simulink model "bus_hvac"  (R2025a)
settings: Solver=VariableStepAuto  StartTime=0.0  StopTime=7200  MaxStep=1  RelTol=1e-3
PreLoadFcn:
  | bus_hvac_params
InitFcn:
  | if ~exist('T_set', 'var'), bus_hvac_params; end
values from neighbouring files (symbols this model uses):
  blow_set = [42 38 28 22]    [bus_hvac_params.m]
  blow_T = [-20 0 10 18]    [bus_hvac_params.m]
  C_cab = cab_mass_factor*rho_air*V_cab*cp_air    (= 361800)    [bus_hvac_params.m]
  c_w = 3600    [bus_hvac_params.m]
  cp_air = 1005    [bus_hvac_params.m]
  d_fan1_off = 0.02    [bus_hvac_params.m]
  d_fan1_on = 0.05    [bus_hvac_params.m]
  d_fan2_off = 0.3    [bus_hvac_params.m]
  d_fan2_on = 0.9    [bus_hvac_params.m]
  d_on = 0.02    [bus_hvac_params.m]
  der_f = [1 1 0.6]    [bus_hvac_params.m]
  der_T = [-40 55 90]    [bus_hvac_params.m]
  e_cool_off = -0.3    [bus_hvac_params.m]
  e_cool_on = 0.5    [bus_hvac_params.m]
  e_heat_off = -0.5    [bus_hvac_params.m]
  e_heat_on = 0.3    [bus_hvac_params.m]
  e_heater_off = -8    [bus_hvac_params.m]
  e_heater_on = 2    [bus_hvac_params.m]
  EER = 2.5    [bus_hvac_params.m]
  eps_front = 0.7    [bus_hvac_params.m]
  front_fan = 1    [bus_hvac_params.m]
  front_margin = 15    [bus_hvac_params.m]
  fuel_enable = 0    [bus_hvac_params.m]
  G_byp = 1/sqrt(K_byp)    [bus_hvac_params.m]
  G_grid = linspace(G_byp, Gc_tab(end) + Gf_tab(end) + G_byp, 30)    [bus_hvac_params.m]
  Gc_tab = 1./sqrt(K_conv + K_valve./h_grid.^2)    [bus_hvac_params.m]
  Gf_tab = 1./sqrt(K_front + K_valve./h_grid.^2)    [bus_hvac_params.m]
  h_grid = linspace(valve_min, 1, 20)    [bus_hvac_params.m]
  hp_COP = [1.6 2.0 2.6 3.2 3.6]    [bus_hvac_params.m]
  hp_enable = 1    [bus_hvac_params.m]
  hp_Qheat = [8000 12000 16000 18000 18000]    [bus_hvac_params.m]
  hp_T = [-20 -10 0 10 20]    [bus_hvac_params.m]
  Ki_cab = 0.004    [bus_hvac_params.m]
  Ki_f = 0.002    [bus_hvac_params.m]
  Ki_h = 0.002    [bus_hvac_params.m]
  Ki_v = 0.0015    [bus_hvac_params.m]
  Kp_f = 0.05    [bus_hvac_params.m]
  Kp_h = 0.08    [bus_hvac_params.m]
  Kp_v = 0.08    [bus_hvac_params.m]
  m_air_front = 0.25    [bus_hvac_params.m]
  M_aux = 8    [bus_hvac_params.m]
  M_conv = 20    [bus_hvac_params.m]
  M_fhx = 1.5    [bus_hvac_params.m]
  m_flow_min = 0.05    [bus_hvac_params.m]
  m_fresh = 0.10    (= 0.1)    [bus_hvac_params.m]
  M_fret = 4    [bus_hvac_params.m]
  M_fsup = 4    [bus_hvac_params.m]
  M_heater = 3    [bus_hvac_params.m]
  mar = [15 10 5]    [bus_hvac_params.m]
  mar_T = [-20 0 15]    [bus_hvac_params.m]
  mtot_tab = sqrt(dp0./(b_pump + K_src + 1./G_grid.^2))    [bus_hvac_params.m]
  n_pass = 20    [bus_hvac_params.m]
  P_fuel_max = 30000    [bus_hvac_params.m]
  P_heater_max = 20000    [bus_hvac_params.m]
  P_pump = 150    [bus_hvac_params.m]
  Q_cool_max = 20000    [bus_hvac_params.m]
  q_pass = 75    [bus_hvac_params.m]
  Q_solar = 0    [bus_hvac_params.m]
  T_cab0 = -10    [bus_hvac_params.m]
  T_conv_max = 65    [bus_hvac_params.m]
  T_cool_lock = 12    [bus_hvac_params.m]
  t_dwell = 300    [bus_hvac_params.m]
  T_fan_off = 35    [bus_hvac_params.m]
  T_fan_on = 40    [bus_hvac_params.m]
  T_fuel_cut = 85    [bus_hvac_params.m]
  t_fuel_ignite = 60    [bus_hvac_params.m]
  T_fuel_off = 78    [bus_hvac_params.m]
  T_fuel_on = 65    [bus_hvac_params.m]
  T_fuel_out_max = 5    [bus_hvac_params.m]
  T_heat_lock = 18    [bus_hvac_params.m]
  T_heater_cut = 88    [bus_hvac_params.m]
  T_heater_cut_hyst = 10    [bus_hvac_params.m]
  t_heater_delay = 10    [bus_hvac_params.m]
  T_out_time = [0 7200]    [bus_hvac_params.m]
  T_out_val = [-10 -10]    [bus_hvac_params.m]
  t_pump_run = 60    [bus_hvac_params.m]
  T_set = 22    [bus_hvac_params.m]
  T_sup_max = 85    [bus_hvac_params.m]
  T_w0 = -10    [bus_hvac_params.m]
  tau_fuel = 60    [bus_hvac_params.m]
  Ts_mode = 5    [bus_hvac_params.m]
  UA_cab = U_wall*A_wall + U_glass*A_glass    (= 222.4)    [bus_hvac_params.m]
  UA_conv_stage = [30 130 220]    [bus_hvac_params.m]
  valve_min = 0.05    [bus_hvac_params.m]
undefined symbols (not defined in the file or in its folder): Kp_cab
settings Model: Creator=giray  LastModifiedBy=giray

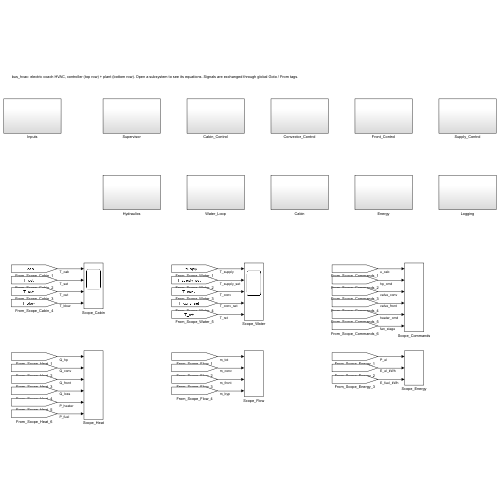
[thumbnail: Simulink's stored preview of the top-level diagram]
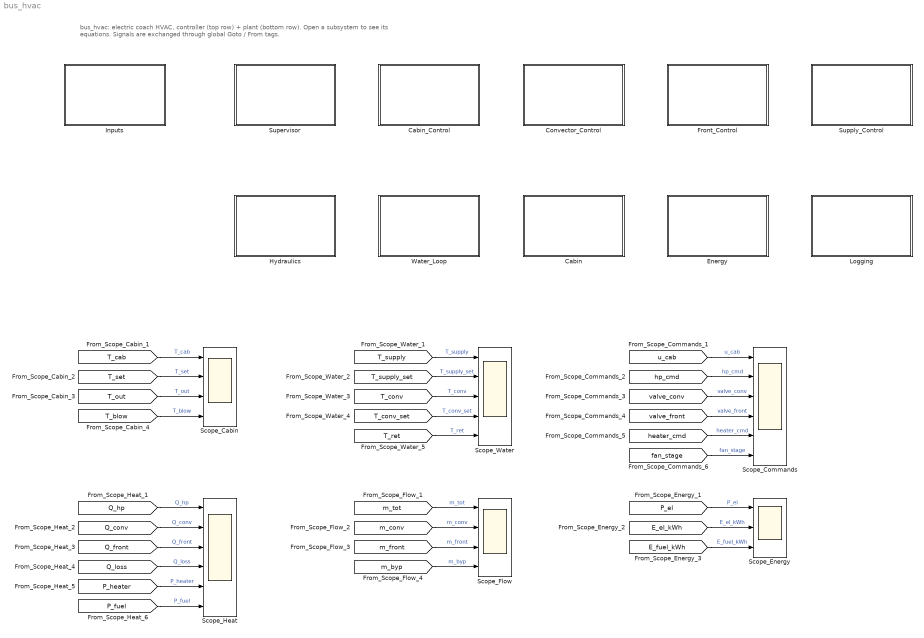
== system bus_hvac ==
  note: bus_hvac: electric coach HVAC, controller (top row) + plant (bottom row). Open a subsystem to see its equations. Signals are exchanged through global Goto / From tags.
  Cabin : Subsystem
  Cabin_Control : Subsystem
  Convector_Control : Subsystem
  Energy : Subsystem
  Front_Control : Subsystem
  Hydraulics : Subsystem
  Inputs : Subsystem
  Logging : Subsystem
  Scope_Cabin : Scope  NumInputPorts=4
  Scope_Commands : Scope  NumInputPorts=6
  Scope_Energy : Scope  NumInputPorts=3
  Scope_Flow : Scope  NumInputPorts=4
  Scope_Heat : Scope  NumInputPorts=6
  Scope_Water : Scope  NumInputPorts=5
  Supervisor : Subsystem
  Supply_Control : Subsystem
  Water_Loop : Subsystem
  wires:
  [T_cab] -> Scope_Cabin/1  "T_cab"
  [T_set] -> Scope_Cabin/2  "T_set"
  [T_out] -> Scope_Cabin/3  "T_out"
  [T_blow] -> Scope_Cabin/4  "T_blow"
  [T_supply] -> Scope_Water/1  "T_supply"
  [T_supply_set] -> Scope_Water/2  "T_supply_set"
  [T_conv] -> Scope_Water/3  "T_conv"
  [T_conv_set] -> Scope_Water/4  "T_conv_set"
  [T_ret] -> Scope_Water/5  "T_ret"
  [u_cab] -> Scope_Commands/1  "u_cab"
  [hp_cmd] -> Scope_Commands/2  "hp_cmd"
  [valve_conv] -> Scope_Commands/3  "valve_conv"
  [valve_front] -> Scope_Commands/4  "valve_front"
  [heater_cmd] -> Scope_Commands/5  "heater_cmd"
  [fan_stage] -> Scope_Commands/6  "fan_stage"
  [Q_hp] -> Scope_Heat/1  "Q_hp"
  [Q_conv] -> Scope_Heat/2  "Q_conv"
  [Q_front] -> Scope_Heat/3  "Q_front"
  [Q_loss] -> Scope_Heat/4  "Q_loss"
  [P_heater] -> Scope_Heat/5  "P_heater"
  [P_fuel] -> Scope_Heat/6  "P_fuel"
  [m_tot] -> Scope_Flow/1  "m_tot"
  [m_conv] -> Scope_Flow/2  "m_conv"
  [m_front] -> Scope_Flow/3  "m_front"
  [m_byp] -> Scope_Flow/4  "m_byp"
  [P_el] -> Scope_Energy/1  "P_el"
  [E_el_kWh] -> Scope_Energy/2  "E_el_kWh"
  [E_fuel_kWh] -> Scope_Energy/3  "E_fuel_kWh"

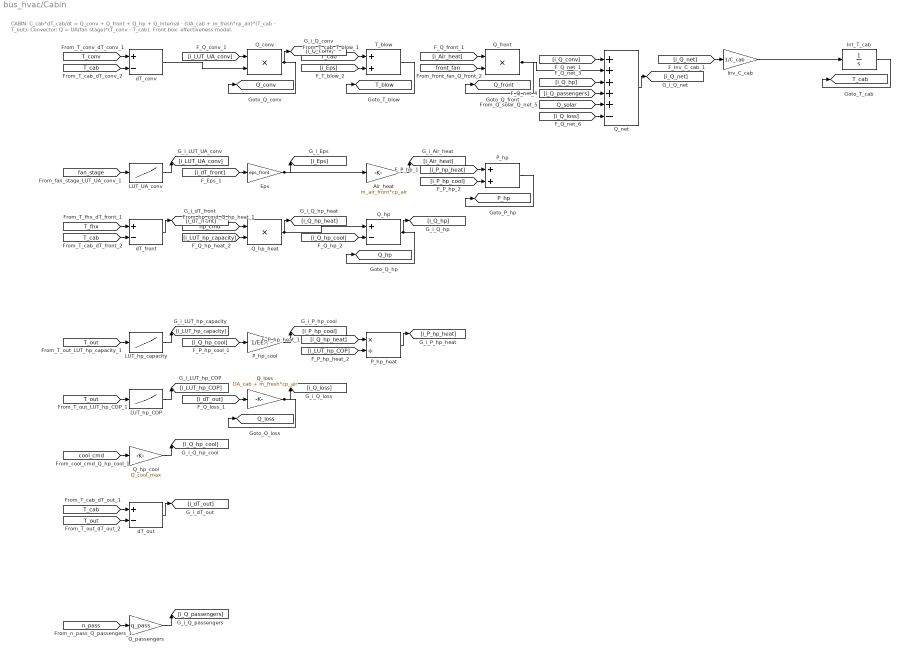
== system bus_hvac/Cabin ==
  note: CABIN: C_cab*dT_cab/dt = Q_conv + Q_front + Q_hp + Q_internal - (UA_cab + m_fresh*cp_air)*(T_cab - T_out). Convector: Q = UA(fan stage)*(T_conv - T_cab). Front box: effectiveness model.
  Air_heat : Gain  Gain=m_air_front*cp_air
  Eps : Gain  Gain=eps_front
  Int_T_cab : Integrator  InitialCondition=T_cab0
  Inv_C_cab : Gain  Gain=1/C_cab
  LUT_UA_conv : Lookup_n-D  NumberOfTableDimensions=1  BreakpointsForDimension1=[0 1 2]  Table=UA_conv_stage  ExtrapMethod=Clip  InternalRulePriority=Speed  RndMeth=Simplest
  LUT_hp_COP : Lookup_n-D  NumberOfTableDimensions=1  BreakpointsForDimension1=hp_T  Table=hp_COP  ExtrapMethod=Clip  InternalRulePriority=Speed  RndMeth=Simplest
  LUT_hp_capacity : Lookup_n-D  NumberOfTableDimensions=1  BreakpointsForDimension1=hp_T  Table=hp_Qheat  ExtrapMethod=Clip  InternalRulePriority=Speed  RndMeth=Simplest
  P_hp : Sum
  P_hp_cool : Gain  Gain=1/EER
  P_hp_heat : Product  Inputs=*/
  Q_conv : Product
  Q_front : Product
  Q_hp : Sum  Inputs=+-
  Q_hp_cool : Gain  Gain=Q_cool_max
  Q_hp_heat : Product
  Q_loss : Gain  Gain=UA_cab + m_fresh*cp_air
  Q_net : Sum  Inputs=+++++-
  Q_passengers : Gain  Gain=q_pass
  T_blow : Sum
  dT_conv : Sum  Inputs=+-
  dT_front : Sum  Inputs=+-
  dT_out : Sum  Inputs=+-
  tag scope: P_hp=global, Q_conv=global, Q_front=global, Q_hp=global, Q_loss=global, T_blow=global, T_cab=global
  wires:
  [T_conv] -> dT_conv/1
  [T_cab] -> dT_conv/2
  [fan_stage] -> LUT_UA_conv/1
  LUT_UA_conv/1 -> [i_LUT_UA_conv]
  [i_LUT_UA_conv] -> Q_conv/1
  dT_conv/1 -> Q_conv/2
  [T_fhx] -> dT_front/1
  [T_cab] -> dT_front/2
  dT_front/1 -> [i_dT_front]
  [i_dT_front] -> Eps/1
  [T_cab] -> T_blow/1
  Eps/1 -> [i_Eps], Air_heat/1
  [i_Eps] -> T_blow/2
  Air_heat/1 -> [i_Air_heat]
  [i_Air_heat] -> Q_front/1
  [front_fan] -> Q_front/2
  [T_out] -> LUT_hp_capacity/1
  [T_out] -> LUT_hp_COP/1
  [hp_cmd] -> Q_hp_heat/1
  LUT_hp_capacity/1 -> [i_LUT_hp_capacity]
  [i_LUT_hp_capacity] -> Q_hp_heat/2
  [cool_cmd] -> Q_hp_cool/1
  Q_hp_heat/1 -> Q_hp/1, [i_Q_hp_heat]
  Q_hp_cool/1 -> [i_Q_hp_cool]
  [i_Q_hp_cool] -> Q_hp/2
  [i_Q_hp_heat] -> P_hp_heat/1
  LUT_hp_COP/1 -> [i_LUT_hp_COP]
  [i_LUT_hp_COP] -> P_hp_heat/2
  [i_Q_hp_cool] -> P_hp_cool/1
  P_hp_heat/1 -> [i_P_hp_heat]
  [i_P_hp_heat] -> P_hp/1
  P_hp_cool/1 -> [i_P_hp_cool]
  [i_P_hp_cool] -> P_hp/2
  [T_cab] -> dT_out/1
  [T_out] -> dT_out/2
  dT_out/1 -> [i_dT_out]
  [i_dT_out] -> Q_loss/1
  [n_pass] -> Q_passengers/1
  Q_conv/1 -> [i_Q_conv], [Q_conv]
  [i_Q_conv] -> Q_net/1
  Q_front/1 -> Q_net/2, [Q_front]
  Q_hp/1 -> [i_Q_hp], [Q_hp]
  [i_Q_hp] -> Q_net/3
  Q_passengers/1 -> [i_Q_passengers]
  [i_Q_passengers] -> Q_net/4
  [Q_solar] -> Q_net/5
  Q_loss/1 -> [i_Q_loss], [Q_loss]
  [i_Q_loss] -> Q_net/6
  Q_net/1 -> [i_Q_net]
  [i_Q_net] -> Inv_C_cab/1
  Inv_C_cab/1 -> Int_T_cab/1
  T_blow/1 -> [T_blow]
  P_hp/1 -> [P_hp]
  Int_T_cab/1 -> [T_cab]

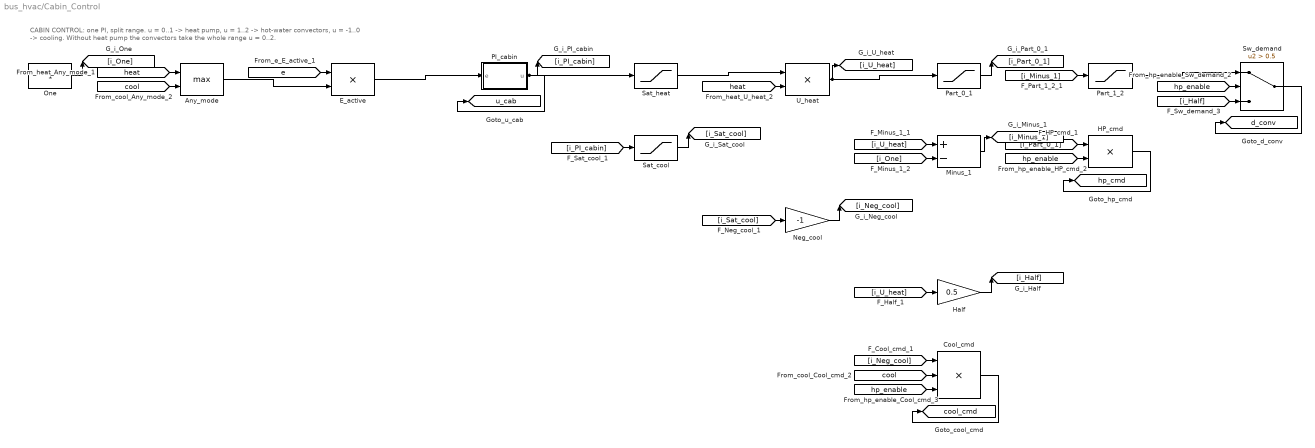
== system bus_hvac/Cabin_Control ==
  note: CABIN CONTROL: one PI, split range. u = 0..1 -> heat pump, u = 1..2 -> hot-water convectors, u = -1..0 -> cooling. Without heat pump the convectors take the whole range u = 0..2.
  Any_mode : MinMax  Function=max  Inputs=2
  Cool_cmd : Product  Inputs=3
  E_active : Product
  HP_cmd : Product
  Half : Gain  Gain=0.5
  Minus_1 : Sum  Inputs=+-
  Neg_cool : Gain  Gain=-1
  One : Constant
  PI_cabin : Subsystem
  Part_0_1 : Saturate  UpperLimit=1  LowerLimit=0
  Part_1_2 : Saturate  UpperLimit=1  LowerLimit=0
  Sat_cool : Saturate  UpperLimit=0  LowerLimit=-1
  Sat_heat : Saturate  UpperLimit=2  LowerLimit=0
  Sw_demand : Switch  Criteria=u2 > Threshold  Threshold=0.5  SaturateOnIntegerOverflow=off  InputSameDT=off
  U_heat : Product
  tag scope: cool_cmd=global, d_conv=global, hp_cmd=global, u_cab=global
  wires:
  [heat] -> Any_mode/1
  [cool] -> Any_mode/2
  [e] -> E_active/1
  Any_mode/1 -> E_active/2
  E_active/1 -> PI_cabin/1(e)
  PI_cabin/1(u) -> Sat_heat/1, [i_PI_cabin], [u_cab]
  Sat_heat/1 -> U_heat/1
  [heat] -> U_heat/2
  U_heat/1 -> Part_0_1/1, [i_U_heat]
  [i_U_heat] -> Minus_1/1
  One/1 -> [i_One]
  [i_One] -> Minus_1/2
  Minus_1/1 -> [i_Minus_1]
  [i_Minus_1] -> Part_1_2/1
  Part_0_1/1 -> [i_Part_0_1]
  [i_Part_0_1] -> HP_cmd/1
  [hp_enable] -> HP_cmd/2
  [i_U_heat] -> Half/1
  Part_1_2/1 -> Sw_demand/1
  [hp_enable] -> Sw_demand/2
  Half/1 -> [i_Half]
  [i_Half] -> Sw_demand/3
  [i_PI_cabin] -> Sat_cool/1
  Sat_cool/1 -> [i_Sat_cool]
  [i_Sat_cool] -> Neg_cool/1
  Neg_cool/1 -> [i_Neg_cool]
  [i_Neg_cool] -> Cool_cmd/1
  [cool] -> Cool_cmd/2
  [hp_enable] -> Cool_cmd/3
  HP_cmd/1 -> [hp_cmd]
  Sw_demand/1 -> [d_conv]
  Cool_cmd/1 -> [cool_cmd]

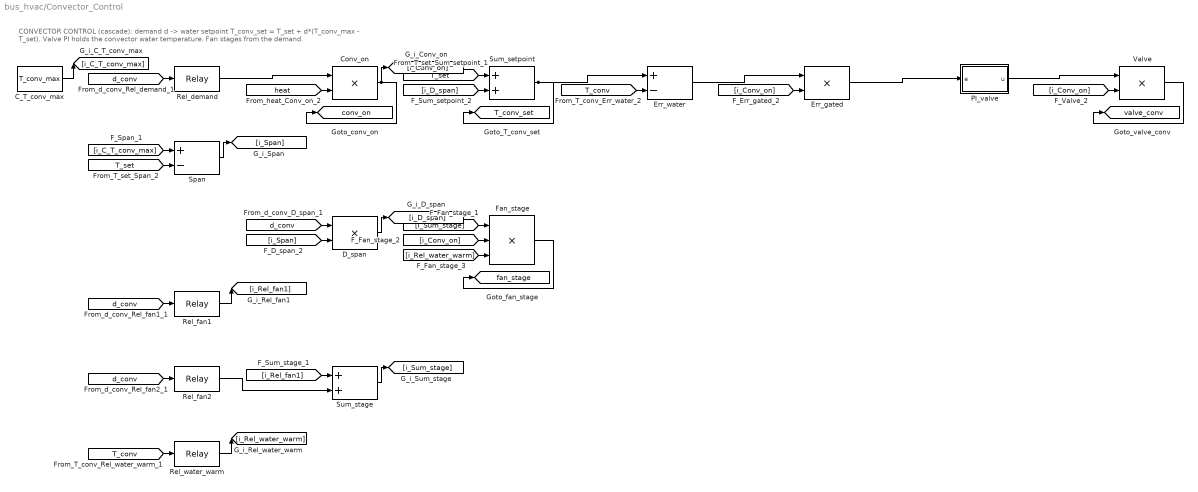
== system bus_hvac/Convector_Control ==
  note: CONVECTOR CONTROL (cascade): demand d -> water setpoint T_conv_set = T_set + d*(T_conv_max - T_set). Valve PI holds the convector water temperature. Fan stages from the demand.
  C_T_conv_max : Constant  Value=T_conv_max
  Conv_on : Product
  D_span : Product
  Err_gated : Product
  Err_water : Sum  Inputs=+-
  Fan_stage : Product  Inputs=3
  PI_valve : Subsystem
  Rel_demand : Relay  OnSwitchValue=d_on  OffSwitchValue=d_on/2
  Rel_fan1 : Relay  OnSwitchValue=d_fan1_on  OffSwitchValue=d_fan1_off
  Rel_fan2 : Relay  OnSwitchValue=d_fan2_on  OffSwitchValue=d_fan2_off
  Rel_water_warm : Relay  OnSwitchValue=T_fan_on  OffSwitchValue=T_fan_off
  Span : Sum  Inputs=+-
  Sum_setpoint : Sum
  Sum_stage : Sum
  Valve : Product
  tag scope: T_conv_set=global, conv_on=global, fan_stage=global, valve_conv=global
  wires:
  [d_conv] -> Rel_demand/1
  Rel_demand/1 -> Conv_on/1
  [heat] -> Conv_on/2
  C_T_conv_max/1 -> [i_C_T_conv_max]
  [i_C_T_conv_max] -> Span/1
  [T_set] -> Span/2
  [d_conv] -> D_span/1
  Span/1 -> [i_Span]
  [i_Span] -> D_span/2
  [T_set] -> Sum_setpoint/1
  D_span/1 -> [i_D_span]
  [i_D_span] -> Sum_setpoint/2
  Sum_setpoint/1 -> Err_water/1, [T_conv_set]
  [T_conv] -> Err_water/2
  Err_water/1 -> Err_gated/1
  Conv_on/1 -> [i_Conv_on], [conv_on]
  [i_Conv_on] -> Err_gated/2
  Err_gated/1 -> PI_valve/1(e)
  PI_valve/1(u) -> Valve/1
  [i_Conv_on] -> Valve/2
  [d_conv] -> Rel_fan1/1
  [d_conv] -> Rel_fan2/1
  Rel_fan1/1 -> [i_Rel_fan1]
  [i_Rel_fan1] -> Sum_stage/1
  Rel_fan2/1 -> Sum_stage/2
  [T_conv] -> Rel_water_warm/1
  Sum_stage/1 -> [i_Sum_stage]
  [i_Sum_stage] -> Fan_stage/1
  [i_Conv_on] -> Fan_stage/2
  Rel_water_warm/1 -> [i_Rel_water_warm]
  [i_Rel_water_warm] -> Fan_stage/3
  Valve/1 -> [valve_conv]
  Fan_stage/1 -> [fan_stage]

== system bus_hvac/Energy ==
  note: ENERGY: electric power = water heater + heat pump compressor + pump. Integrated to kWh.
  E_el : Integrator
  E_fuel : Integrator
  P_el : Sum  Inputs=+++
  P_pump_el : Gain  Gain=P_pump
  To_kWh_el : Gain  Gain=1/3.6e6
  To_kWh_fuel : Gain  Gain=1/3.6e6
  tag scope: E_el_kWh=global, E_fuel_kWh=global, P_el=global
  wires:
  [pump_cmd] -> P_pump_el/1
  [P_heater] -> P_el/1
  [P_hp] -> P_el/2
  P_pump_el/1 -> P_el/3
  P_el/1 -> To_kWh_el/1, [P_el]
  To_kWh_el/1 -> E_el/1
  [P_fuel] -> To_kWh_fuel/1
  To_kWh_fuel/1 -> [i_To_kWh_fuel]
  [i_To_kWh_fuel] -> E_fuel/1
  E_el/1 -> [E_el_kWh]
  E_fuel/1 -> [E_fuel_kWh]

== system bus_hvac/Front_Control ==
  note: FRONT BOX CONTROL: blow-out temperature setpoint from the outdoor temperature. Valve PI holds the blow-out temperature.
  Err_blow : Sum  Inputs=+-
  Err_gated : Product
  Front_on : Product
  LUT_blow_set : Lookup_n-D  NumberOfTableDimensions=1  BreakpointsForDimension1=blow_T  Table=blow_set  ExtrapMethod=Clip  InternalRulePriority=Speed  RndMeth=Simplest
  PI_valve : Subsystem
  Valve : Product
  tag scope: T_blow_set=global, front_on=global, valve_front=global
  wires:
  [heat] -> Front_on/1
  [front_fan] -> Front_on/2
  [T_out] -> LUT_blow_set/1
  LUT_blow_set/1 -> [i_LUT_blow_set], [T_blow_set]
  [i_LUT_blow_set] -> Err_blow/1
  [T_blow] -> Err_blow/2
  Err_blow/1 -> Err_gated/1
  Front_on/1 -> [i_Front_on], [front_on]
  [i_Front_on] -> Err_gated/2
  Err_gated/1 -> PI_valve/1(e)
  PI_valve/1(u) -> Valve/1
  [i_Front_on] -> Valve/2
  Valve/1 -> [valve_front]

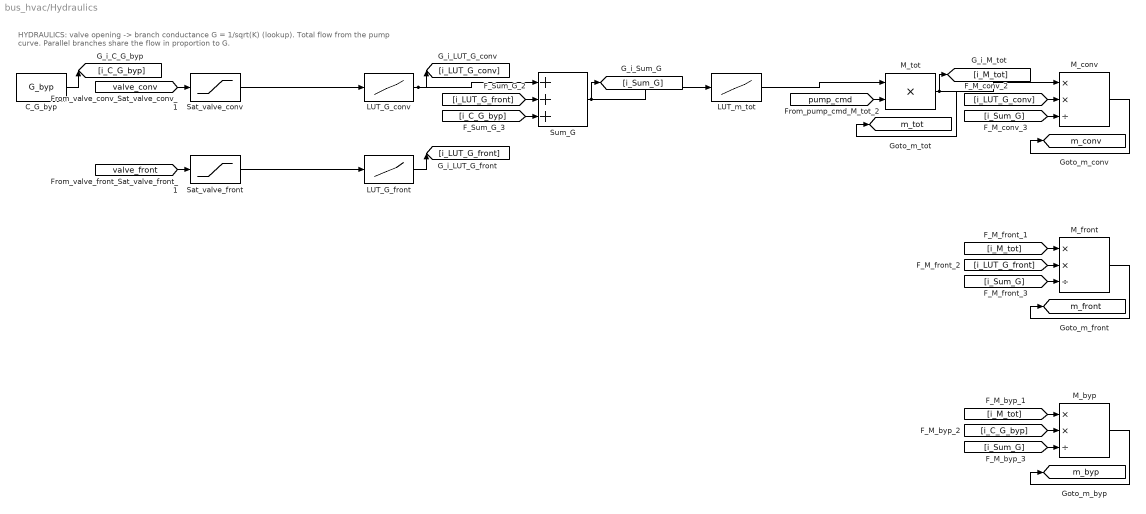
== system bus_hvac/Hydraulics ==
  note: HYDRAULICS: valve opening -> branch conductance G = 1/sqrt(K) (lookup). Total flow from the pump curve. Parallel branches share the flow in proportion to G.
  C_G_byp : Constant  Value=G_byp
  LUT_G_conv : Lookup_n-D  NumberOfTableDimensions=1  BreakpointsForDimension1=h_grid  Table=Gc_tab  ExtrapMethod=Clip  InternalRulePriority=Speed  RndMeth=Simplest
  LUT_G_front : Lookup_n-D  NumberOfTableDimensions=1  BreakpointsForDimension1=h_grid  Table=Gf_tab  ExtrapMethod=Clip  InternalRulePriority=Speed  RndMeth=Simplest
  LUT_m_tot : Lookup_n-D  NumberOfTableDimensions=1  BreakpointsForDimension1=G_grid  Table=mtot_tab  ExtrapMethod=Clip  InternalRulePriority=Speed  RndMeth=Simplest
  M_byp : Product  Inputs=**/
  M_conv : Product  Inputs=**/
  M_front : Product  Inputs=**/
  M_tot : Product
  Sat_valve_conv : Saturate  UpperLimit=1  LowerLimit=valve_min
  Sat_valve_front : Saturate  UpperLimit=1  LowerLimit=valve_min
  Sum_G : Sum  Inputs=+++
  tag scope: m_byp=global, m_conv=global, m_front=global, m_tot=global
  wires:
  [valve_conv] -> Sat_valve_conv/1
  Sat_valve_conv/1 -> LUT_G_conv/1
  [valve_front] -> Sat_valve_front/1
  Sat_valve_front/1 -> LUT_G_front/1
  LUT_G_conv/1 -> Sum_G/1, [i_LUT_G_conv]
  LUT_G_front/1 -> [i_LUT_G_front]
  [i_LUT_G_front] -> Sum_G/2
  C_G_byp/1 -> [i_C_G_byp]
  [i_C_G_byp] -> Sum_G/3
  Sum_G/1 -> LUT_m_tot/1, [i_Sum_G]
  LUT_m_tot/1 -> M_tot/1
  [pump_cmd] -> M_tot/2
  M_tot/1 -> M_conv/1, [i_M_tot], [m_tot]
  [i_LUT_G_conv] -> M_conv/2
  [i_Sum_G] -> M_conv/3
  [i_M_tot] -> M_front/1
  [i_LUT_G_front] -> M_front/2
  [i_Sum_G] -> M_front/3
  [i_M_tot] -> M_byp/1
  [i_C_G_byp] -> M_byp/2
  [i_Sum_G] -> M_byp/3
  M_conv/1 -> [m_conv]
  M_front/1 -> [m_front]
  M_byp/1 -> [m_byp]

== system bus_hvac/Inputs ==
  note: INPUTS: scenario values and the outdoor temperature profile (T_out_time, T_out_val).
  C_Q_solar : Constant  Value=Q_solar
  C_T_set : Constant  Value=T_set
  C_front_fan : Constant  Value=front_fan
  C_fuel_enable : Constant  Value=fuel_enable
  C_hp_enable : Constant  Value=hp_enable
  C_n_pass : Constant  Value=n_pass
  Clock : Clock
  Profile_T_out : Lookup_n-D  NumberOfTableDimensions=1  BreakpointsForDimension1=T_out_time  Table=T_out_val  ExtrapMethod=Clip  InternalRulePriority=Speed  RndMeth=Simplest
  tag scope: Q_solar=global, T_out=global, T_set=global, front_fan=global, fuel_enable=global, hp_enable=global, n_pass=global
  wires:
  Clock/1 -> [i_Clock]
  [i_Clock] -> Profile_T_out/1
  C_T_set/1 -> [T_set]
  C_n_pass/1 -> [n_pass]
  C_Q_solar/1 -> [Q_solar]
  C_hp_enable/1 -> [hp_enable]
  C_fuel_enable/1 -> [fuel_enable]
  C_front_fan/1 -> [front_fan]
  Profile_T_out/1 -> [T_out]

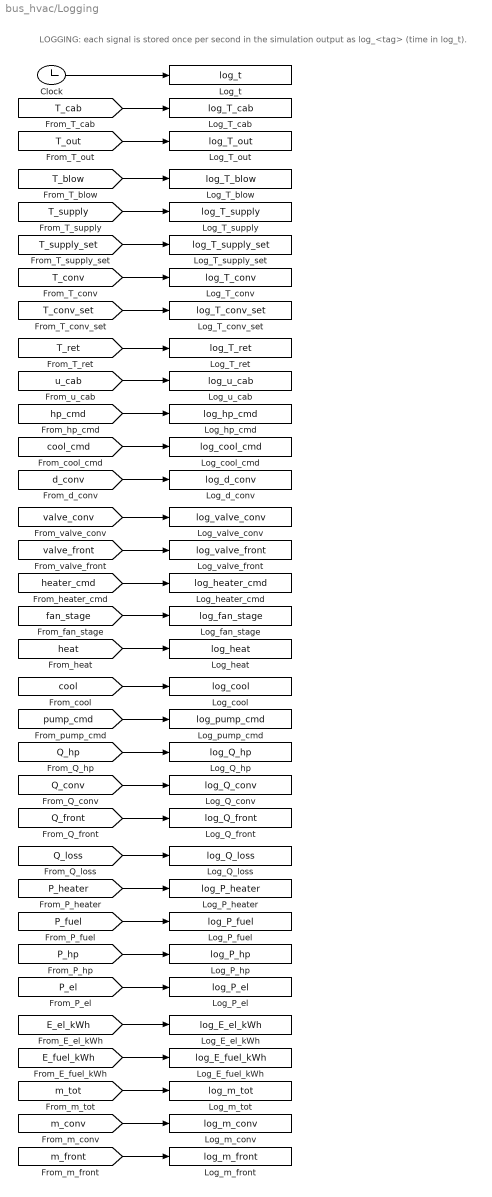
== system bus_hvac/Logging ==
  note: LOGGING: each signal is stored once per second in the simulation output as log_<tag> (time in log_t).
  Clock : Clock
  Log_E_el_kWh : ToWorkspace  VariableName=log_E_el_kWh  SampleTime=1
  Log_E_fuel_kWh : ToWorkspace  VariableName=log_E_fuel_kWh  SampleTime=1
  Log_P_el : ToWorkspace  VariableName=log_P_el  SampleTime=1
  Log_P_fuel : ToWorkspace  VariableName=log_P_fuel  SampleTime=1
  Log_P_heater : ToWorkspace  VariableName=log_P_heater  SampleTime=1
  Log_P_hp : ToWorkspace  VariableName=log_P_hp  SampleTime=1
  Log_Q_conv : ToWorkspace  VariableName=log_Q_conv  SampleTime=1
  Log_Q_front : ToWorkspace  VariableName=log_Q_front  SampleTime=1
  Log_Q_hp : ToWorkspace  VariableName=log_Q_hp  SampleTime=1
  Log_Q_loss : ToWorkspace  VariableName=log_Q_loss  SampleTime=1
  Log_T_blow : ToWorkspace  VariableName=log_T_blow  SampleTime=1
  Log_T_cab : ToWorkspace  VariableName=log_T_cab  SampleTime=1
  Log_T_conv : ToWorkspace  VariableName=log_T_conv  SampleTime=1
  Log_T_conv_set : ToWorkspace  VariableName=log_T_conv_set  SampleTime=1
  Log_T_out : ToWorkspace  VariableName=log_T_out  SampleTime=1
  Log_T_ret : ToWorkspace  VariableName=log_T_ret  SampleTime=1
  Log_T_supply : ToWorkspace  VariableName=log_T_supply  SampleTime=1
  Log_T_supply_set : ToWorkspace  VariableName=log_T_supply_set  SampleTime=1
  Log_cool : ToWorkspace  VariableName=log_cool  SampleTime=1
  Log_cool_cmd : ToWorkspace  VariableName=log_cool_cmd  SampleTime=1
  Log_d_conv : ToWorkspace  VariableName=log_d_conv  SampleTime=1
  Log_fan_stage : ToWorkspace  VariableName=log_fan_stage  SampleTime=1
  Log_heat : ToWorkspace  VariableName=log_heat  SampleTime=1
  Log_heater_cmd : ToWorkspace  VariableName=log_heater_cmd  SampleTime=1
  Log_hp_cmd : ToWorkspace  VariableName=log_hp_cmd  SampleTime=1
  Log_m_conv : ToWorkspace  VariableName=log_m_conv  SampleTime=1
  Log_m_front : ToWorkspace  VariableName=log_m_front  SampleTime=1
  Log_m_tot : ToWorkspace  VariableName=log_m_tot  SampleTime=1
  Log_pump_cmd : ToWorkspace  VariableName=log_pump_cmd  SampleTime=1
  Log_t : ToWorkspace  VariableName=log_t  SampleTime=1
  Log_u_cab : ToWorkspace  VariableName=log_u_cab  SampleTime=1
  Log_valve_conv : ToWorkspace  VariableName=log_valve_conv  SampleTime=1
  Log_valve_front : ToWorkspace  VariableName=log_valve_front  SampleTime=1
  wires:
  Clock/1 -> Log_t/1
  [T_cab] -> Log_T_cab/1
  [T_out] -> Log_T_out/1
  [T_blow] -> Log_T_blow/1
  [T_supply] -> Log_T_supply/1
  [T_supply_set] -> Log_T_supply_set/1
  [T_conv] -> Log_T_conv/1
  [T_conv_set] -> Log_T_conv_set/1
  [T_ret] -> Log_T_ret/1
  [u_cab] -> Log_u_cab/1
  [hp_cmd] -> Log_hp_cmd/1
  [cool_cmd] -> Log_cool_cmd/1
  [d_conv] -> Log_d_conv/1
  [valve_conv] -> Log_valve_conv/1
  [valve_front] -> Log_valve_front/1
  [heater_cmd] -> Log_heater_cmd/1
  [fan_stage] -> Log_fan_stage/1
  [heat] -> Log_heat/1
  [cool] -> Log_cool/1
  [pump_cmd] -> Log_pump_cmd/1
  [Q_hp] -> Log_Q_hp/1
  [Q_conv] -> Log_Q_conv/1
  [Q_front] -> Log_Q_front/1
  [Q_loss] -> Log_Q_loss/1
  [P_heater] -> Log_P_heater/1
  [P_fuel] -> Log_P_fuel/1
  [P_hp] -> Log_P_hp/1
  [P_el] -> Log_P_el/1
  [E_el_kWh] -> Log_E_el_kWh/1
  [E_fuel_kWh] -> Log_E_fuel_kWh/1
  [m_tot] -> Log_m_tot/1
  [m_conv] -> Log_m_conv/1
  [m_front] -> Log_m_front/1

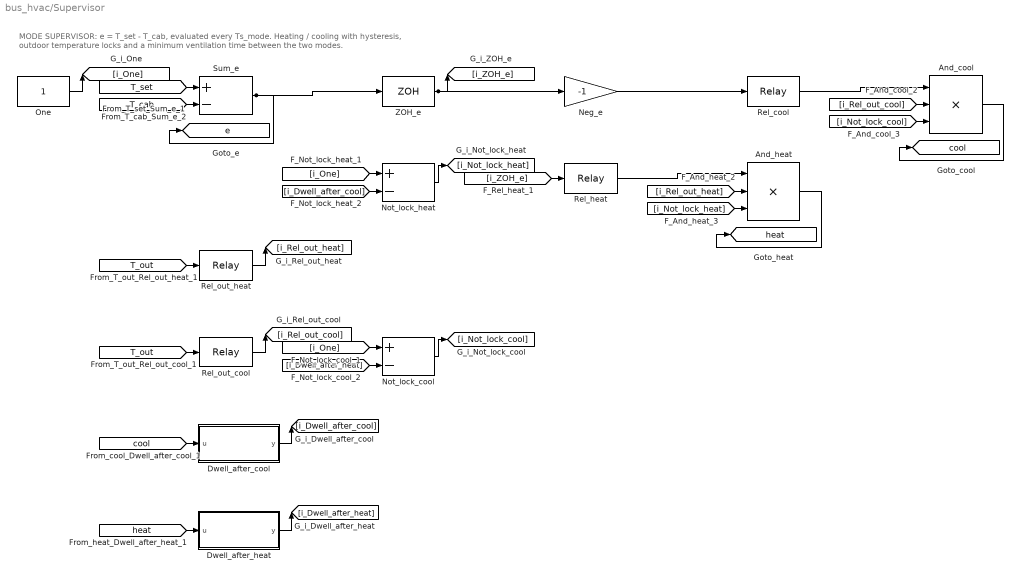
== system bus_hvac/Supervisor ==
  note: MODE SUPERVISOR: e = T_set - T_cab, evaluated every Ts_mode. Heating / cooling with hysteresis, outdoor temperature locks and a minimum ventilation time between the two modes.
  And_cool : Product  Inputs=3
  And_heat : Product  Inputs=3
  Dwell_after_cool : Subsystem
  Dwell_after_heat : Subsystem
  Neg_e : Gain  Gain=-1
  Not_lock_cool : Sum  Inputs=+-
  Not_lock_heat : Sum  Inputs=+-
  One : Constant
  Rel_cool : Relay  OnSwitchValue=e_cool_on  OffSwitchValue=e_cool_off
  Rel_heat : Relay  OnSwitchValue=e_heat_on  OffSwitchValue=e_heat_off
  Rel_out_cool : Relay  OnSwitchValue=T_cool_lock+2  OffSwitchValue=T_cool_lock
  Rel_out_heat : Relay  OnSwitchValue=T_heat_lock  OffSwitchValue=T_heat_lock-2  OnOutputValue=0  OffOutputValue=1
  Sum_e : Sum  Inputs=+-
  ZOH_e : ZeroOrderHold  SampleTime=Ts_mode
  tag scope: cool=global, e=global, heat=global
  wires:
  [T_set] -> Sum_e/1
  [T_cab] -> Sum_e/2
  Sum_e/1 -> ZOH_e/1, [e]
  ZOH_e/1 -> Neg_e/1, [i_ZOH_e]
  [i_ZOH_e] -> Rel_heat/1
  Neg_e/1 -> Rel_cool/1
  [T_out] -> Rel_out_heat/1
  [T_out] -> Rel_out_cool/1
  [cool] -> Dwell_after_cool/1(u)
  [heat] -> Dwell_after_heat/1(u)
  One/1 -> [i_One]
  [i_One] -> Not_lock_heat/1
  Dwell_after_cool/1(y) -> [i_Dwell_after_cool]
  [i_Dwell_after_cool] -> Not_lock_heat/2
  [i_One] -> Not_lock_cool/1
  Dwell_after_heat/1(y) -> [i_Dwell_after_heat]
  [i_Dwell_after_heat] -> Not_lock_cool/2
  Rel_heat/1 -> And_heat/1
  Rel_out_heat/1 -> [i_Rel_out_heat]
  [i_Rel_out_heat] -> And_heat/2
  Not_lock_heat/1 -> [i_Not_lock_heat]
  [i_Not_lock_heat] -> And_heat/3
  Rel_cool/1 -> And_cool/1
  Rel_out_cool/1 -> [i_Rel_out_cool]
  [i_Rel_out_cool] -> And_cool/2
  Not_lock_cool/1 -> [i_Not_lock_cool]
  [i_Not_lock_cool] -> And_cool/3
  And_heat/1 -> [heat]
  And_cool/1 -> [cool]

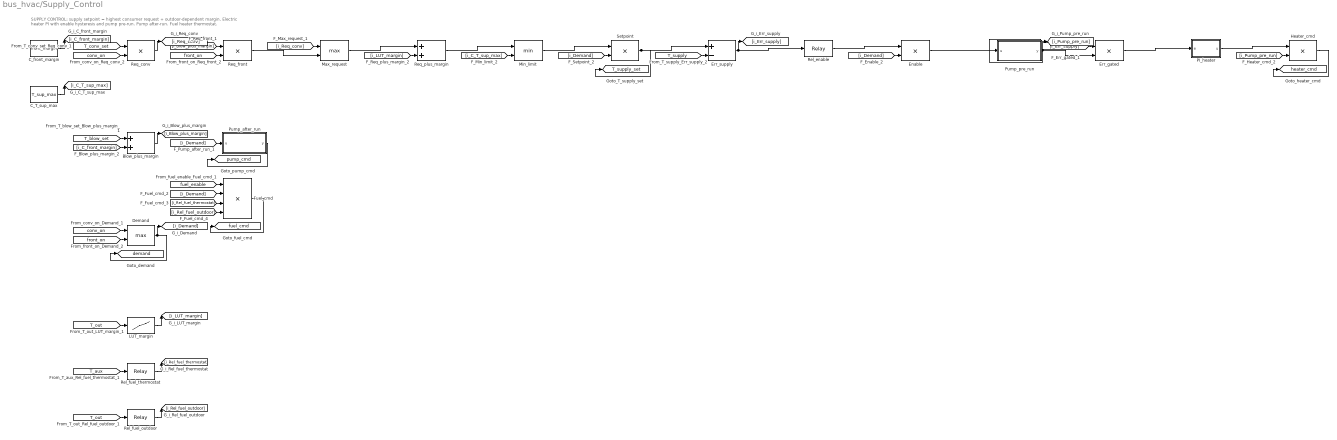
== system bus_hvac/Supply_Control ==
  note: SUPPLY CONTROL: supply setpoint = highest consumer request + outdoor-dependent margin. Electric heater PI with enable hysteresis and pump pre-run. Pump after-run. Fuel heater thermostat.
  Blow_plus_margin : Sum
  C_T_sup_max : Constant  Value=T_sup_max
  C_front_margin : Constant  Value=front_margin
  Demand : MinMax  Function=max  Inputs=2
  Enable : Product
  Err_gated : Product
  Err_supply : Sum  Inputs=+-
  Fuel_cmd : Product  Inputs=4
  Heater_cmd : Product
  LUT_margin : Lookup_n-D  NumberOfTableDimensions=1  BreakpointsForDimension1=mar_T  Table=mar  ExtrapMethod=Clip  InternalRulePriority=Speed  RndMeth=Simplest
  Max_request : MinMax  Function=max  Inputs=2
  Min_limit : MinMax  Inputs=2
  PI_heater : Subsystem
  Pump_after_run : Subsystem
  Pump_pre_run : Subsystem
  Rel_enable : Relay  OnSwitchValue=e_heater_on  OffSwitchValue=e_heater_off
  Rel_fuel_outdoor : Relay  OnSwitchValue=T_fuel_out_max  OffSwitchValue=T_fuel_out_max-2  OnOutputValue=0  OffOutputValue=1
  Rel_fuel_thermostat : Relay  OnSwitchValue=T_fuel_off  OffSwitchValue=T_fuel_on  OnOutputValue=0  OffOutputValue=1
  Req_conv : Product
  Req_front : Product
  Req_plus_margin : Sum
  Setpoint : Product
  tag scope: T_supply_set=global, demand=global, fuel_cmd=global, heater_cmd=global, pump_cmd=global
  wires:
  [T_conv_set] -> Req_conv/1
  [conv_on] -> Req_conv/2
  [T_blow_set] -> Blow_plus_margin/1
  C_front_margin/1 -> [i_C_front_margin]
  [i_C_front_margin] -> Blow_plus_margin/2
  Blow_plus_margin/1 -> [i_Blow_plus_margin]
  [i_Blow_plus_margin] -> Req_front/1
  [front_on] -> Req_front/2
  Req_conv/1 -> [i_Req_conv]
  [i_Req_conv] -> Max_request/1
  Req_front/1 -> Max_request/2
  [conv_on] -> Demand/1
  [front_on] -> Demand/2
  [T_out] -> LUT_margin/1
  Max_request/1 -> Req_plus_margin/1
  LUT_margin/1 -> [i_LUT_margin]
  [i_LUT_margin] -> Req_plus_margin/2
  Req_plus_margin/1 -> Min_limit/1
  C_T_sup_max/1 -> [i_C_T_sup_max]
  [i_C_T_sup_max] -> Min_limit/2
  Min_limit/1 -> Setpoint/1
  Demand/1 -> [i_Demand], [demand]
  [i_Demand] -> Setpoint/2
  [i_Demand] -> Pump_after_run/1(u)
  Setpoint/1 -> Err_supply/1, [T_supply_set]
  [T_supply] -> Err_supply/2
  Err_supply/1 -> Rel_enable/1, [i_Err_supply]
  Rel_enable/1 -> Enable/1
  [i_Demand] -> Enable/2
  Enable/1 -> Pump_pre_run/1(u)
  [i_Err_supply] -> Err_gated/1
  Pump_pre_run/1(y) -> Err_gated/2, [i_Pump_pre_run]
  Err_gated/1 -> PI_heater/1(e)
  PI_heater/1(u) -> Heater_cmd/1
  [i_Pump_pre_run] -> Heater_cmd/2
  [T_aux] -> Rel_fuel_thermostat/1
  [T_out] -> Rel_fuel_outdoor/1
  [fuel_enable] -> Fuel_cmd/1
  [i_Demand] -> Fuel_cmd/2
  Rel_fuel_thermostat/1 -> [i_Rel_fuel_thermostat]
  [i_Rel_fuel_thermostat] -> Fuel_cmd/3
  Rel_fuel_outdoor/1 -> [i_Rel_fuel_outdoor]
  [i_Rel_fuel_outdoor] -> Fuel_cmd/4
  Pump_after_run/1(y) -> [pump_cmd]
  Heater_cmd/1 -> [heater_cmd]
  Fuel_cmd/1 -> [fuel_cmd]

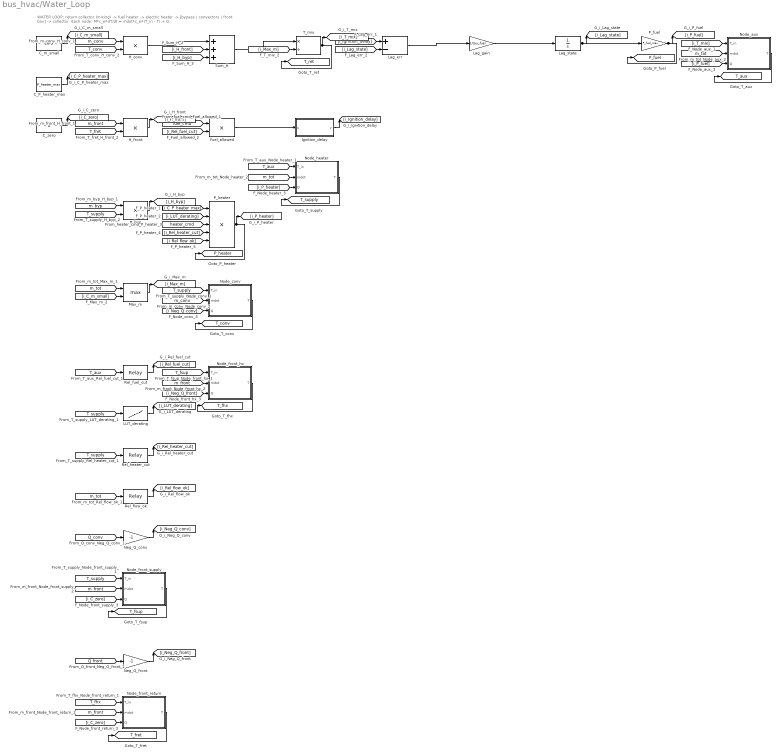
== system bus_hvac/Water_Loop ==
  note: WATER LOOP: return collector (mixing) -> fuel heater -> electric heater -> [bypass | convectors | front box] -> collector. Each node: M*c_w*dT/dt = mdot*c_w*(T_in - T) + Q.
  C_P_heater_max : Constant  Value=P_heater_max
  C_m_small : Constant  Value=1e-3
  C_zero : Constant  Value=0
  Fuel_allowed : Product
  H_byp : Product
  H_conv : Product
  H_front : Product
  Ignition_delay : Subsystem
  LUT_derating : Lookup_n-D  NumberOfTableDimensions=1  BreakpointsForDimension1=der_T  Table=der_f  ExtrapMethod=Clip  InternalRulePriority=Speed  RndMeth=Simplest
  Lag_err : Sum  Inputs=+-
  Lag_gain : Gain  Gain=1/tau_fuel
  Lag_state : Integrator
  Max_m : MinMax  Function=max  Inputs=2
  Neg_Q_conv : Gain  Gain=-1
  Neg_Q_front : Gain  Gain=-1
  Node_aux : Subsystem
  Node_conv : Subsystem
  Node_front_hx : Subsystem
  Node_front_return : Subsystem
  Node_front_supply : Subsystem
  Node_heater : Subsystem
  P_fuel : Gain  Gain=P_fuel_max
  P_heater : Product  Inputs=5
  Rel_flow_ok : Relay  OnSwitchValue=m_flow_min  OffSwitchValue=m_flow_min/2
  Rel_fuel_cut : Relay  OnSwitchValue=T_fuel_cut  OffSwitchValue=T_fuel_cut-10  OnOutputValue=0  OffOutputValue=1
  Rel_heater_cut : Relay  OnSwitchValue=T_heater_cut  OffSwitchValue=T_heater_cut-T_heater_cut_hyst  OnOutputValue=0  OffOutputValue=1
  Sum_H : Sum  Inputs=+++
  T_mix : Product  Inputs=*/
  tag scope: P_fuel=global, P_heater=global, T_aux=global, T_conv=global, T_fhx=global, T_fret=global, T_fsup=global, T_ret=global, T_supply=global
  wires:
  [m_conv] -> H_conv/1
  [T_conv] -> H_conv/2
  [m_front] -> H_front/1
  [T_fret] -> H_front/2
  [m_byp] -> H_byp/1
  [T_supply] -> H_byp/2
  H_conv/1 -> Sum_H/1
  H_front/1 -> [i_H_front]
  [i_H_front] -> Sum_H/2
  H_byp/1 -> [i_H_byp]
  [i_H_byp] -> Sum_H/3
  [m_tot] -> Max_m/1
  C_m_small/1 -> [i_C_m_small]
  [i_C_m_small] -> Max_m/2
  Sum_H/1 -> T_mix/1
  Max_m/1 -> [i_Max_m]
  [i_Max_m] -> T_mix/2
  [T_aux] -> Rel_fuel_cut/1
  [fuel_cmd] -> Fuel_allowed/1
  Rel_fuel_cut/1 -> [i_Rel_fuel_cut]
  [i_Rel_fuel_cut] -> Fuel_allowed/2
  Fuel_allowed/1 -> Ignition_delay/1(u)
  Ignition_delay/1(y) -> [i_Ignition_delay]
  [i_Ignition_delay] -> Lag_err/1
  Lag_state/1 -> [i_Lag_state], P_fuel/1
  [i_Lag_state] -> Lag_err/2
  Lag_err/1 -> Lag_gain/1
  Lag_gain/1 -> Lag_state/1
  T_mix/1 -> [i_T_mix], [T_ret]
  [i_T_mix] -> Node_aux/1(T_in)
  [m_tot] -> Node_aux/2(mdot)
  P_fuel/1 -> [i_P_fuel], [P_fuel]
  [i_P_fuel] -> Node_aux/3(Q)
  [T_supply] -> LUT_derating/1
  [T_supply] -> Rel_heater_cut/1
  [m_tot] -> Rel_flow_ok/1
  C_P_heater_max/1 -> [i_C_P_heater_max]
  [i_C_P_heater_max] -> P_heater/1
  LUT_derating/1 -> [i_LUT_derating]
  [i_LUT_derating] -> P_heater/2
  [heater_cmd] -> P_heater/3
  Rel_heater_cut/1 -> [i_Rel_heater_cut]
  [i_Rel_heater_cut] -> P_heater/4
  Rel_flow_ok/1 -> [i_Rel_flow_ok]
  [i_Rel_flow_ok] -> P_heater/5
  [T_aux] -> Node_heater/1(T_in)
  [m_tot] -> Node_heater/2(mdot)
  P_heater/1 -> [i_P_heater], [P_heater]
  [i_P_heater] -> Node_heater/3(Q)
  [Q_conv] -> Neg_Q_conv/1
  [T_supply] -> Node_conv/1(T_in)
  [m_conv] -> Node_conv/2(mdot)
  Neg_Q_conv/1 -> [i_Neg_Q_conv]
  [i_Neg_Q_conv] -> Node_conv/3(Q)
  [T_supply] -> Node_front_supply/1(T_in)
  [m_front] -> Node_front_supply/2(mdot)
  C_zero/1 -> [i_C_zero]
  [i_C_zero] -> Node_front_supply/3(Q)
  [Q_front] -> Neg_Q_front/1
  [T_fsup] -> Node_front_hx/1(T_in)
  [m_front] -> Node_front_hx/2(mdot)
  Neg_Q_front/1 -> [i_Neg_Q_front]
  [i_Neg_Q_front] -> Node_front_hx/3(Q)
  [T_fhx] -> Node_front_return/1(T_in)
  [m_front] -> Node_front_return/2(mdot)
  [i_C_zero] -> Node_front_return/3(Q)
  Node_aux/1(T) -> [T_aux]
  Node_heater/1(T) -> [T_supply]
  Node_conv/1(T) -> [T_conv]
  Node_front_supply/1(T) -> [T_fsup]
  Node_front_hx/1(T) -> [T_fhx]
  Node_front_return/1(T) -> [T_fret]

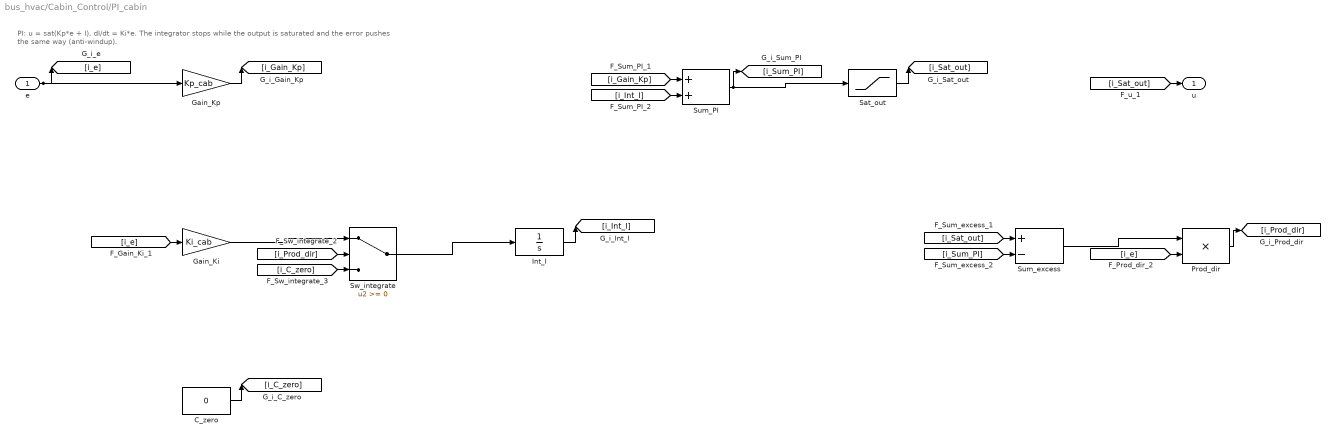
== system bus_hvac/Cabin_Control/PI_cabin ==
  note: PI: u = sat(Kp*e + I), dI/dt = Ki*e. The integrator stops while the output is saturated and the error pushes the same way (anti-windup).
  e : Inport
  C_zero : Constant  Value=0
  Gain_Ki : Gain  Gain=Ki_cab
  Gain_Kp : Gain  Gain=Kp_cab
  Int_I : Integrator
  Prod_dir : Product
  Sat_out : Saturate  UpperLimit=2  LowerLimit=-1
  Sum_PI : Sum
  Sum_excess : Sum  Inputs=+-
  Sw_integrate : Switch  SaturateOnIntegerOverflow=off  InputSameDT=off
  u : Outport
  wires:
  e/1 -> Gain_Kp/1, [i_e]
  [i_e] -> Gain_Ki/1
  Gain_Ki/1 -> Sw_integrate/1
  Prod_dir/1 -> [i_Prod_dir]
  [i_Prod_dir] -> Sw_integrate/2
  C_zero/1 -> [i_C_zero]
  [i_C_zero] -> Sw_integrate/3
  Sw_integrate/1 -> Int_I/1
  Gain_Kp/1 -> [i_Gain_Kp]
  [i_Gain_Kp] -> Sum_PI/1
  Int_I/1 -> [i_Int_I]
  [i_Int_I] -> Sum_PI/2
  Sum_PI/1 -> Sat_out/1, [i_Sum_PI]
  Sat_out/1 -> [i_Sat_out]
  [i_Sat_out] -> Sum_excess/1
  [i_Sum_PI] -> Sum_excess/2
  Sum_excess/1 -> Prod_dir/1
  [i_e] -> Prod_dir/2
  [i_Sat_out] -> u/1

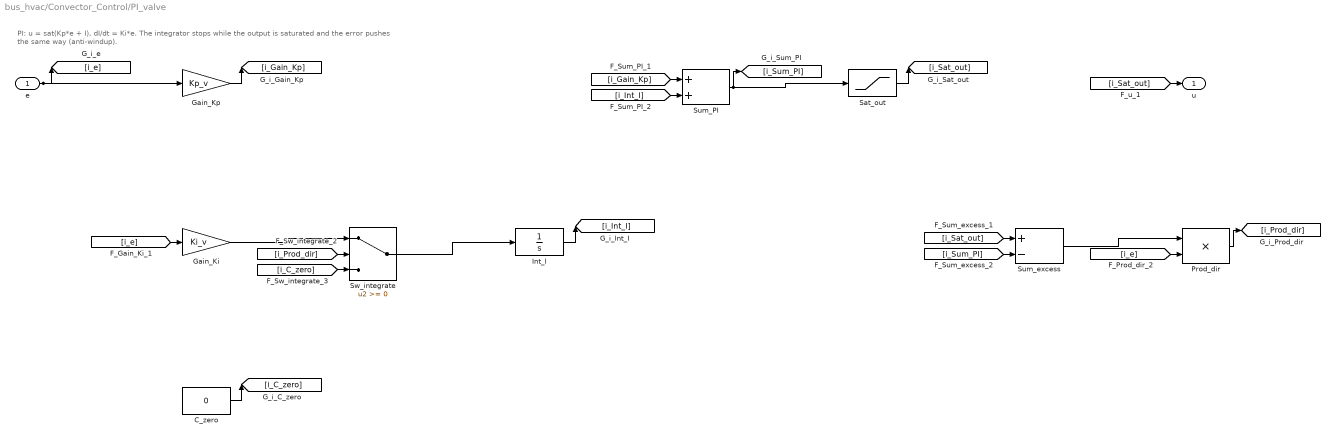
== system bus_hvac/Convector_Control/PI_valve ==
  note: PI: u = sat(Kp*e + I), dI/dt = Ki*e. The integrator stops while the output is saturated and the error pushes the same way (anti-windup).
  e : Inport
  C_zero : Constant  Value=0
  Gain_Ki : Gain  Gain=Ki_v
  Gain_Kp : Gain  Gain=Kp_v
  Int_I : Integrator
  Prod_dir : Product
  Sat_out : Saturate  UpperLimit=1  LowerLimit=0
  Sum_PI : Sum
  Sum_excess : Sum  Inputs=+-
  Sw_integrate : Switch  SaturateOnIntegerOverflow=off  InputSameDT=off
  u : Outport
  wires:
  e/1 -> Gain_Kp/1, [i_e]
  [i_e] -> Gain_Ki/1
  Gain_Ki/1 -> Sw_integrate/1
  Prod_dir/1 -> [i_Prod_dir]
  [i_Prod_dir] -> Sw_integrate/2
  C_zero/1 -> [i_C_zero]
  [i_C_zero] -> Sw_integrate/3
  Sw_integrate/1 -> Int_I/1
  Gain_Kp/1 -> [i_Gain_Kp]
  [i_Gain_Kp] -> Sum_PI/1
  Int_I/1 -> [i_Int_I]
  [i_Int_I] -> Sum_PI/2
  Sum_PI/1 -> Sat_out/1, [i_Sum_PI]
  Sat_out/1 -> [i_Sat_out]
  [i_Sat_out] -> Sum_excess/1
  [i_Sum_PI] -> Sum_excess/2
  Sum_excess/1 -> Prod_dir/1
  [i_e] -> Prod_dir/2
  [i_Sat_out] -> u/1

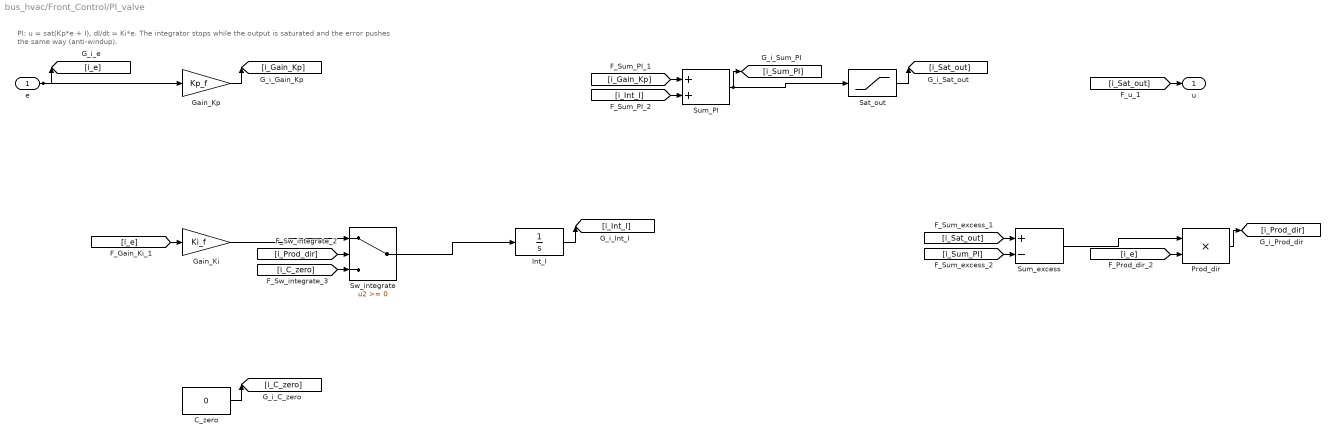
== system bus_hvac/Front_Control/PI_valve ==
  note: PI: u = sat(Kp*e + I), dI/dt = Ki*e. The integrator stops while the output is saturated and the error pushes the same way (anti-windup).
  e : Inport
  C_zero : Constant  Value=0
  Gain_Ki : Gain  Gain=Ki_f
  Gain_Kp : Gain  Gain=Kp_f
  Int_I : Integrator
  Prod_dir : Product
  Sat_out : Saturate  UpperLimit=1  LowerLimit=0
  Sum_PI : Sum
  Sum_excess : Sum  Inputs=+-
  Sw_integrate : Switch  SaturateOnIntegerOverflow=off  InputSameDT=off
  u : Outport
  wires:
  e/1 -> Gain_Kp/1, [i_e]
  [i_e] -> Gain_Ki/1
  Gain_Ki/1 -> Sw_integrate/1
  Prod_dir/1 -> [i_Prod_dir]
  [i_Prod_dir] -> Sw_integrate/2
  C_zero/1 -> [i_C_zero]
  [i_C_zero] -> Sw_integrate/3
  Sw_integrate/1 -> Int_I/1
  Gain_Kp/1 -> [i_Gain_Kp]
  [i_Gain_Kp] -> Sum_PI/1
  Int_I/1 -> [i_Int_I]
  [i_Int_I] -> Sum_PI/2
  Sum_PI/1 -> Sat_out/1, [i_Sum_PI]
  Sat_out/1 -> [i_Sat_out]
  [i_Sat_out] -> Sum_excess/1
  [i_Sum_PI] -> Sum_excess/2
  Sum_excess/1 -> Prod_dir/1
  [i_e] -> Prod_dir/2
  [i_Sat_out] -> u/1

== system bus_hvac/Supervisor/Dwell_after_cool ==
  note: OFF-DELAY: after the input drops to 0 the output stays 1 for a while (down-counter).
  u : Inport
  C_step : Constant
  C_time : Constant  Value=t_dwell
  Remaining : UnitDelay  HasFrameUpgradeWarning=on
  Sat_0_1 : Saturate  UpperLimit=1  LowerLimit=0
  Sat_zero : Saturate  UpperLimit=inf  LowerLimit=0
  Sum_count : Sum  Inputs=+-
  Sw_load : Switch  Criteria=u2 > Threshold  Threshold=0.5  SaturateOnIntegerOverflow=off  InputSameDT=off
  y : Outport
  wires:
  C_time/1 -> Sw_load/1
  u/1 -> [i_u]
  [i_u] -> Sw_load/2
  Sat_zero/1 -> [i_Sat_zero]
  [i_Sat_zero] -> Sw_load/3
  Sw_load/1 -> Remaining/1
  Remaining/1 -> Sum_count/1, [i_Remaining]
  C_step/1 -> [i_C_step]
  [i_C_step] -> Sum_count/2
  Sum_count/1 -> Sat_zero/1
  [i_Remaining] -> Sat_0_1/1
  Sat_0_1/1 -> [i_Sat_0_1]
  [i_Sat_0_1] -> y/1

== system bus_hvac/Supervisor/Dwell_after_heat ==
  note: OFF-DELAY: after the input drops to 0 the output stays 1 for a while (down-counter).
  u : Inport
  C_step : Constant
  C_time : Constant  Value=t_dwell
  Remaining : UnitDelay  HasFrameUpgradeWarning=on
  Sat_0_1 : Saturate  UpperLimit=1  LowerLimit=0
  Sat_zero : Saturate  UpperLimit=inf  LowerLimit=0
  Sum_count : Sum  Inputs=+-
  Sw_load : Switch  Criteria=u2 > Threshold  Threshold=0.5  SaturateOnIntegerOverflow=off  InputSameDT=off
  y : Outport
  wires:
  C_time/1 -> Sw_load/1
  u/1 -> [i_u]
  [i_u] -> Sw_load/2
  Sat_zero/1 -> [i_Sat_zero]
  [i_Sat_zero] -> Sw_load/3
  Sw_load/1 -> Remaining/1
  Remaining/1 -> Sum_count/1, [i_Remaining]
  C_step/1 -> [i_C_step]
  [i_C_step] -> Sum_count/2
  Sum_count/1 -> Sat_zero/1
  [i_Remaining] -> Sat_0_1/1
  Sat_0_1/1 -> [i_Sat_0_1]
  [i_Sat_0_1] -> y/1

== system bus_hvac/Supply_Control/PI_heater ==
  note: PI: u = sat(Kp*e + I), dI/dt = Ki*e. The integrator stops while the output is saturated and the error pushes the same way (anti-windup).
  e : Inport
  C_zero : Constant  Value=0
  Gain_Ki : Gain  Gain=Ki_h
  Gain_Kp : Gain  Gain=Kp_h
  Int_I : Integrator
  Prod_dir : Product
  Sat_out : Saturate  UpperLimit=1  LowerLimit=0
  Sum_PI : Sum
  Sum_excess : Sum  Inputs=+-
  Sw_integrate : Switch  SaturateOnIntegerOverflow=off  InputSameDT=off
  u : Outport
  wires:
  e/1 -> Gain_Kp/1, [i_e]
  [i_e] -> Gain_Ki/1
  Gain_Ki/1 -> Sw_integrate/1
  Prod_dir/1 -> [i_Prod_dir]
  [i_Prod_dir] -> Sw_integrate/2
  C_zero/1 -> [i_C_zero]
  [i_C_zero] -> Sw_integrate/3
  Sw_integrate/1 -> Int_I/1
  Gain_Kp/1 -> [i_Gain_Kp]
  [i_Gain_Kp] -> Sum_PI/1
  Int_I/1 -> [i_Int_I]
  [i_Int_I] -> Sum_PI/2
  Sum_PI/1 -> Sat_out/1, [i_Sum_PI]
  Sat_out/1 -> [i_Sat_out]
  [i_Sat_out] -> Sum_excess/1
  [i_Sum_PI] -> Sum_excess/2
  Sum_excess/1 -> Prod_dir/1
  [i_e] -> Prod_dir/2
  [i_Sat_out] -> u/1

== system bus_hvac/Supply_Control/Pump_after_run ==
  note: OFF-DELAY: after the input drops to 0 the output stays 1 for a while (down-counter).
  u : Inport
  C_step : Constant
  C_time : Constant  Value=t_pump_run
  Max_out : MinMax  Function=max  Inputs=2
  Remaining : UnitDelay  HasFrameUpgradeWarning=on
  Sat_0_1 : Saturate  UpperLimit=1  LowerLimit=0
  Sat_zero : Saturate  UpperLimit=inf  LowerLimit=0
  Sum_count : Sum  Inputs=+-
  Sw_load : Switch  Criteria=u2 > Threshold  Threshold=0.5  SaturateOnIntegerOverflow=off  InputSameDT=off
  y : Outport
  wires:
  C_time/1 -> Sw_load/1
  u/1 -> [i_u]
  [i_u] -> Sw_load/2
  Sat_zero/1 -> [i_Sat_zero]
  [i_Sat_zero] -> Sw_load/3
  Sw_load/1 -> Remaining/1, [i_Sw_load]
  Remaining/1 -> Sum_count/1
  C_step/1 -> [i_C_step]
  [i_C_step] -> Sum_count/2
  Sum_count/1 -> Sat_zero/1
  [i_Sw_load] -> Sat_0_1/1
  [i_u] -> Max_out/1
  Sat_0_1/1 -> Max_out/2
  Max_out/1 -> [i_Max_out]
  [i_Max_out] -> y/1

== system bus_hvac/Supply_Control/Pump_pre_run ==
  note: ON-DELAY: the output becomes 1 only after the input has been 1 for a while without interruption (up-counter).
  u : Inport
  C_step : Constant
  C_zero : Constant  Value=0
  Counter : UnitDelay  HasFrameUpgradeWarning=on
  Prod_out : Product
  Rel_done : Relay  OnSwitchValue=(t_heater_delay)-0.5  OffSwitchValue=(t_heater_delay)-0.5
  Sat_time : Saturate  UpperLimit=t_heater_delay  LowerLimit=0
  Sum_count : Sum
  Sw_count : Switch  Criteria=u2 > Threshold  Threshold=0.5  SaturateOnIntegerOverflow=off  InputSameDT=off
  y : Outport
  wires:
  Counter/1 -> Sum_count/1
  C_step/1 -> [i_C_step]
  [i_C_step] -> Sum_count/2
  Sum_count/1 -> Sat_time/1
  Sat_time/1 -> Sw_count/1
  u/1 -> [i_u]
  [i_u] -> Sw_count/2
  C_zero/1 -> [i_C_zero]
  [i_C_zero] -> Sw_count/3
  Sw_count/1 -> [i_Sw_count], Rel_done/1
  [i_Sw_count] -> Counter/1
  Rel_done/1 -> Prod_out/1
  [i_u] -> Prod_out/2
  Prod_out/1 -> y/1

== system bus_hvac/Water_Loop/Ignition_delay ==
  note: ON-DELAY: the output becomes 1 only after the input has been 1 for a while without interruption (up-counter).
  u : Inport
  C_step : Constant
  C_zero : Constant  Value=0
  Counter : UnitDelay  HasFrameUpgradeWarning=on
  Prod_out : Product
  Rel_done : Relay  OnSwitchValue=(t_fuel_ignite)-0.5  OffSwitchValue=(t_fuel_ignite)-0.5
  Sat_time : Saturate  UpperLimit=t_fuel_ignite  LowerLimit=0
  Sum_count : Sum
  Sw_count : Switch  Criteria=u2 > Threshold  Threshold=0.5  SaturateOnIntegerOverflow=off  InputSameDT=off
  y : Outport
  wires:
  Counter/1 -> Sum_count/1
  C_step/1 -> [i_C_step]
  [i_C_step] -> Sum_count/2
  Sum_count/1 -> Sat_time/1
  Sat_time/1 -> Sw_count/1
  u/1 -> [i_u]
  [i_u] -> Sw_count/2
  C_zero/1 -> [i_C_zero]
  [i_C_zero] -> Sw_count/3
  Sw_count/1 -> [i_Sw_count], Rel_done/1
  [i_Sw_count] -> Counter/1
  Rel_done/1 -> Prod_out/1
  [i_u] -> Prod_out/2
  Prod_out/1 -> y/1

== system bus_hvac/Water_Loop/Node_aux ==
  note: WATER NODE: mass * c_w * dT/dt = mdot * c_w * (T_in - T) + Q
  T_in : Inport
  mdot : Inport  Port=2
  Q : Inport  Port=3
  Gain_1_Mc : Gain  Gain=1/((M_aux)*c_w)
  Gain_c_w : Gain  Gain=c_w
  Int_T : Integrator  InitialCondition=T_w0
  Prod_flow : Product
  Sum_dT : Sum  Inputs=+-
  Sum_net : Sum
  T : Outport
  wires:
  T_in/1 -> Sum_dT/1
  Int_T/1 -> [i_Int_T], T/1
  [i_Int_T] -> Sum_dT/2
  Sum_dT/1 -> Prod_flow/1
  mdot/1 -> [i_mdot]
  [i_mdot] -> Prod_flow/2
  Prod_flow/1 -> Gain_c_w/1
  Gain_c_w/1 -> Sum_net/1
  Q/1 -> [i_Q]
  [i_Q] -> Sum_net/2
  Sum_net/1 -> Gain_1_Mc/1
  Gain_1_Mc/1 -> Int_T/1

== system bus_hvac/Water_Loop/Node_conv ==
  note: WATER NODE: mass * c_w * dT/dt = mdot * c_w * (T_in - T) + Q
  T_in : Inport
  mdot : Inport  Port=2
  Q : Inport  Port=3
  Gain_1_Mc : Gain  Gain=1/((M_conv)*c_w)
  Gain_c_w : Gain  Gain=c_w
  Int_T : Integrator  InitialCondition=T_w0
  Prod_flow : Product
  Sum_dT : Sum  Inputs=+-
  Sum_net : Sum
  T : Outport
  wires:
  T_in/1 -> Sum_dT/1
  Int_T/1 -> [i_Int_T], T/1
  [i_Int_T] -> Sum_dT/2
  Sum_dT/1 -> Prod_flow/1
  mdot/1 -> [i_mdot]
  [i_mdot] -> Prod_flow/2
  Prod_flow/1 -> Gain_c_w/1
  Gain_c_w/1 -> Sum_net/1
  Q/1 -> [i_Q]
  [i_Q] -> Sum_net/2
  Sum_net/1 -> Gain_1_Mc/1
  Gain_1_Mc/1 -> Int_T/1

== system bus_hvac/Water_Loop/Node_front_hx ==
  note: WATER NODE: mass * c_w * dT/dt = mdot * c_w * (T_in - T) + Q
  T_in : Inport
  mdot : Inport  Port=2
  Q : Inport  Port=3
  Gain_1_Mc : Gain  Gain=1/((M_fhx)*c_w)
  Gain_c_w : Gain  Gain=c_w
  Int_T : Integrator  InitialCondition=T_w0
  Prod_flow : Product
  Sum_dT : Sum  Inputs=+-
  Sum_net : Sum
  T : Outport
  wires:
  T_in/1 -> Sum_dT/1
  Int_T/1 -> [i_Int_T], T/1
  [i_Int_T] -> Sum_dT/2
  Sum_dT/1 -> Prod_flow/1
  mdot/1 -> [i_mdot]
  [i_mdot] -> Prod_flow/2
  Prod_flow/1 -> Gain_c_w/1
  Gain_c_w/1 -> Sum_net/1
  Q/1 -> [i_Q]
  [i_Q] -> Sum_net/2
  Sum_net/1 -> Gain_1_Mc/1
  Gain_1_Mc/1 -> Int_T/1

== system bus_hvac/Water_Loop/Node_front_return ==
  note: WATER NODE: mass * c_w * dT/dt = mdot * c_w * (T_in - T) + Q
  T_in : Inport
  mdot : Inport  Port=2
  Q : Inport  Port=3
  Gain_1_Mc : Gain  Gain=1/((M_fret)*c_w)
  Gain_c_w : Gain  Gain=c_w
  Int_T : Integrator  InitialCondition=T_w0
  Prod_flow : Product
  Sum_dT : Sum  Inputs=+-
  Sum_net : Sum
  T : Outport
  wires:
  T_in/1 -> Sum_dT/1
  Int_T/1 -> [i_Int_T], T/1
  [i_Int_T] -> Sum_dT/2
  Sum_dT/1 -> Prod_flow/1
  mdot/1 -> [i_mdot]
  [i_mdot] -> Prod_flow/2
  Prod_flow/1 -> Gain_c_w/1
  Gain_c_w/1 -> Sum_net/1
  Q/1 -> [i_Q]
  [i_Q] -> Sum_net/2
  Sum_net/1 -> Gain_1_Mc/1
  Gain_1_Mc/1 -> Int_T/1

== system bus_hvac/Water_Loop/Node_front_supply ==
  note: WATER NODE: mass * c_w * dT/dt = mdot * c_w * (T_in - T) + Q
  T_in : Inport
  mdot : Inport  Port=2
  Q : Inport  Port=3
  Gain_1_Mc : Gain  Gain=1/((M_fsup)*c_w)
  Gain_c_w : Gain  Gain=c_w
  Int_T : Integrator  InitialCondition=T_w0
  Prod_flow : Product
  Sum_dT : Sum  Inputs=+-
  Sum_net : Sum
  T : Outport
  wires:
  T_in/1 -> Sum_dT/1
  Int_T/1 -> [i_Int_T], T/1
  [i_Int_T] -> Sum_dT/2
  Sum_dT/1 -> Prod_flow/1
  mdot/1 -> [i_mdot]
  [i_mdot] -> Prod_flow/2
  Prod_flow/1 -> Gain_c_w/1
  Gain_c_w/1 -> Sum_net/1
  Q/1 -> [i_Q]
  [i_Q] -> Sum_net/2
  Sum_net/1 -> Gain_1_Mc/1
  Gain_1_Mc/1 -> Int_T/1

== system bus_hvac/Water_Loop/Node_heater ==
  note: WATER NODE: mass * c_w * dT/dt = mdot * c_w * (T_in - T) + Q
  T_in : Inport
  mdot : Inport  Port=2
  Q : Inport  Port=3
  Gain_1_Mc : Gain  Gain=1/((M_heater)*c_w)
  Gain_c_w : Gain  Gain=c_w
  Int_T : Integrator  InitialCondition=T_w0
  Prod_flow : Product
  Sum_dT : Sum  Inputs=+-
  Sum_net : Sum
  T : Outport
  wires:
  T_in/1 -> Sum_dT/1
  Int_T/1 -> [i_Int_T], T/1
  [i_Int_T] -> Sum_dT/2
  Sum_dT/1 -> Prod_flow/1
  mdot/1 -> [i_mdot]
  [i_mdot] -> Prod_flow/2
  Prod_flow/1 -> Gain_c_w/1
  Gain_c_w/1 -> Sum_net/1
  Q/1 -> [i_Q]
  [i_Q] -> Sum_net/2
  Sum_net/1 -> Gain_1_Mc/1
  Gain_1_Mc/1 -> Int_T/1
